simulink model "rect5angles3p"  (Simulink 7.4)
settings: Solver=ode45  StartTime=0.0  StopTime=0.08  RelTol=1e-3
undefined symbols (not defined in the file or in its folder): DiscIntNeverNeededParam, Ts
libraries: powerlib x23, powerlib_extras x1
settings Model: Creator=Safano  LastModifiedBy=ELMAY

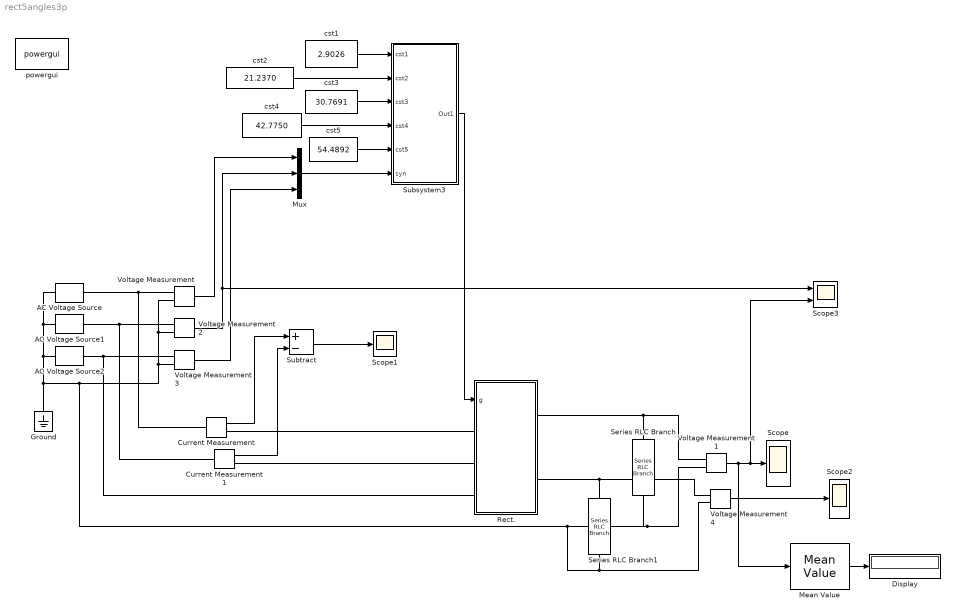
== system rect5angles3p ==
  AC Voltage Source : powerlib/Electrical Sources/AC Voltage Source  DialogController=POWERSYS.PowerSysDialog  SystemSampleTime=-1  Amplitude=220  Phase=0  Frequency=50  SampleTime=0  Measurements=None
  AC Voltage Source1 : powerlib/Electrical Sources/AC Voltage Source  DialogController=POWERSYS.PowerSysDialog  SystemSampleTime=-1  Amplitude=220  Phase=-120  Frequency=50  SampleTime=0  Measurements=None
  AC Voltage Source2 : powerlib/Electrical Sources/AC Voltage Source  DialogController=POWERSYS.PowerSysDialog  SystemSampleTime=-1  Amplitude=220  Phase=+120  Frequency=50  SampleTime=0  Measurements=None
  Current Measurement : powerlib/Measurements/Current Measurement  DialogController=POWERSYS.PowerSysDialog  SystemSampleTime=-1  PhasorSimulation=off  OutputType=Complex  PSBequivalent=0
  Current Measurement1 : powerlib/Measurements/Current Measurement  DialogController=POWERSYS.PowerSysDialog  SystemSampleTime=-1  PhasorSimulation=off  OutputType=Complex  PSBequivalent=0
  Display : Display
  Ground : powerlib/Elements/Ground  DialogController=POWERSYS.PowerSysDialog  PhysicalDomain=powersysdomain  SubClassName=unknown  LeftPortType=p1  RightPortType=p1  LConnTagsString=a
  Mean Value : powerlib_extras/Measurements/Mean Value  DialogController=POWERSYS.PowerSysDialog  SystemSampleTime=-1  Period=1/50
  Mux : Mux  Inputs=3
  Rect. : Subsystem
  Scope : Scope
      settings: SaveName=outrect
  Scope1 : Scope
  Scope2 : Scope
      settings: SaveName=outneg
  Scope3 : Scope  NumInputPorts=2
      settings: YMin=-5~-5  YMax=5~5  SaveName=crt1
  Series RLC Branch : powerlib/Elements/Series RLC Branch  DialogController=POWERSYS.PowerSysDialog  PhysicalDomain=powersysdomain  SubClassName=unknown  LeftPortType=p1  RightPortType=p1  LConnTagsString=__new0  RConnTagsString=__new0  BranchType=R  Resistance=0.3  Inductance=51e-3  SetiL0=off  InitialCurrent=0  Capacitance=1e-6  Setx0=off  InitialVoltage=0  Measurements=None
  Series RLC Branch1 : powerlib/Elements/Series RLC Branch  DialogController=POWERSYS.PowerSysDialog  PhysicalDomain=powersysdomain  SubClassName=unknown  LeftPortType=p1  RightPortType=p1  LConnTagsString=__new0  RConnTagsString=__new0  BranchType=R  Resistance=0.3  Inductance=15e-3  SetiL0=off  InitialCurrent=0  Capacitance=1e-6  Setx0=off  InitialVoltage=0  Measurements=None
  Subsystem3 : Subsystem
  Subtract : Sum  Inputs=+-  OutDataType=fixdt(1, 16)  OutScaling=2^-10
  Voltage Measurement{,1..4} (5 alike) : powerlib/Measurements/Voltage Measurement  DialogController=POWERSYS.PowerSysDialog  SystemSampleTime=-1  PhasorSimulation=off  OutputType=Complex  PSBequivalent=0
  cst1 : Constant  Value=2.9026  OutDataType=fixdt(1, 16)  OutScaling=2^0
  cst2 : Constant  Value=21.2370  OutDataType=fixdt(1, 16)  OutScaling=2^0
  cst3 : Constant  Value=30.7691  OutDataType=fixdt(1, 16)  OutScaling=2^0
  cst4 : Constant  Value=42.7750  OutDataType=fixdt(1, 16)  OutScaling=2^0
  cst5 : Constant  Value=54.4892  OutDataType=fixdt(1, 16)  OutScaling=2^0
  powergui : powerlib/powergui  Priority=1  SystemSampleTime=-1  SimulationMode=Discrete  SampleTime=50e-6  frequency=60  SPID=off  DisableSnubberDevices=off  DisableRonSwitches=off  DisableVfSwitches=off  SwTol=0  Interpol=off  frequencyindice=50  echomessages=off  HookPort=off  DisplayEquations=off  FunctionMessages=off  EnableUseOfTLC=off  x0status=blocks  RestoreLinks=warning  Frange=[0:2:500]  Ylog=off  Xlog=on  ShowGrid=off  save=off  variable=ZData  structure=outneg  ZoomFFT=off  StartTime=0.0  cycles=8  DisplayStyle=1  fundamental=150  FreqAxis=off  MaxFrequency=1000  frequencyindicesteady=1  RmsSteady=1  display=off  Ts=0  methode=off
  wires:
  cst1/1 -> Subsystem3/1(cst1)
  cst2/1 -> Subsystem3/2(cst2)
  cst3/1 -> Subsystem3/3(cst3)
  cst4/1 -> Subsystem3/4(cst4)
  cst5/1 -> Subsystem3/5(cst5)
  Mux/1 -> Subsystem3/6(syn)
  Voltage Measurement/1 -> Mux/1
  Voltage Measurement2/1 -> Mux/2, Scope3/1
  Voltage Measurement3/1 -> Mux/3
  Current Measurement/1 -> Subtract/1
  Current Measurement1/1 -> Subtract/2
  Subtract/1 -> Scope1/1
  Subsystem3/1(Out1) -> Rect./1(g)
  Voltage Measurement1/1 -> Scope/1, Scope3/2, Mean Value/1
  Voltage Measurement4/1 -> Scope2/1
  Mean Value/1 -> Display/1
  connections:
  Voltage Measurement/LConn1 -- AC Voltage Source/RConn1 -- Current Measurement/LConn1
  Voltage Measurement2/LConn1 -- AC Voltage Source1/RConn1 -- Current Measurement1/LConn1
  AC Voltage Source2/RConn1 -- Voltage Measurement3/LConn1 -- Rect./LConn3
  Current Measurement/RConn1 -- Rect./LConn1
  Voltage Measurement4/LConn2 -- Series RLC Branch1/RConn1 -- Voltage Measurement/LConn2 -- Voltage Measurement2/LConn2 -- Voltage Measurement3/LConn2 -- AC Voltage Source/LConn1 -- AC Voltage Source1/LConn1 -- AC Voltage Source2/LConn1 -- Ground/LConn1 -- Voltage Measurement1/LConn2 -- Series RLC Branch/RConn1
  Current Measurement1/RConn1 -- Rect./LConn2
  Rect./RConn1 -- Voltage Measurement1/LConn1 -- Series RLC Branch/LConn1
  Series RLC Branch1/LConn1 -- Rect./RConn2 -- Voltage Measurement4/LConn1

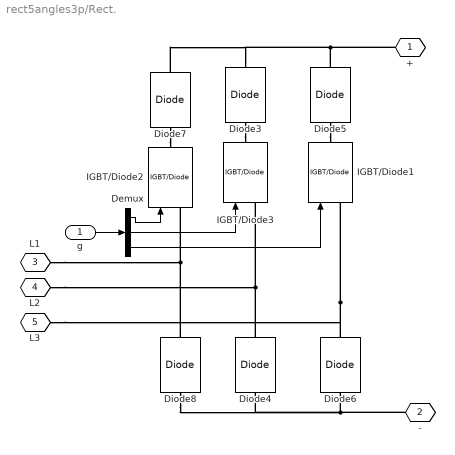
== system rect5angles3p/Rect. ==
  g : Inport  OutDataType=fixdt(1, 16)  OutScaling=2^0
  Demux : Demux  Outputs=3
  Diode{3..8} (6 alike) : powerlib/Power Electronics/Diode  DialogController=POWERSYS.PowerSysDialog  SystemSampleTime=-1  Ron=0.001  Lon=0  Vf=0.8  IC=0  UseSnubber=off  Rs=500  Cs=250e-9  Measurements=off
  IGBT/Diode1 : powerlib/Power Electronics/IGBT//Diode  DialogController=POWERSYS.PowerSysDialog  SystemSampleTime=-1  Ron=1e-3  Rs=1e5  Cs=inf  Measurements=off
  IGBT/Diode2 : powerlib/Power Electronics/IGBT//Diode  DialogController=POWERSYS.PowerSysDialog  SystemSampleTime=-1  Ron=1e-3  Rs=1e5  Cs=inf  Measurements=off
  IGBT/Diode3 : powerlib/Power Electronics/IGBT//Diode  DialogController=POWERSYS.PowerSysDialog  SystemSampleTime=-1  Ron=1e-3  Rs=1e5  Cs=inf  Measurements=off
  + : PMIOPort  Tag=PMCPort  Port=1  Side=Right
  - : PMIOPort  Tag=PMCPort  Port=2  Side=Right
  L1 : PMIOPort  Tag=PMCPort  Port=3  Side=Left
  L2 : PMIOPort  Tag=PMCPort  Port=4  Side=Left
  L3 : PMIOPort  Tag=PMCPort  Port=5  Side=Left
  wires:
  Demux/1 -> IGBT/Diode2/1
  Demux/2 -> IGBT/Diode3/1
  Demux/3 -> IGBT/Diode1/1
  g/1 -> Demux/1
  connections:
  Diode3/LConn1 -- IGBT/Diode3/RConn1
  +/RConn1 -- Diode5/RConn1 -- Diode7/RConn1 -- Diode3/RConn1
  -/RConn1 -- Diode8/LConn1 -- Diode4/LConn1 -- Diode6/LConn1
  L2/RConn1 -- Diode4/RConn1 -- IGBT/Diode3/LConn1
  Diode5/LConn1 -- IGBT/Diode1/RConn1
  L3/RConn1 -- Diode6/RConn1 -- IGBT/Diode1/LConn1
  Diode7/LConn1 -- IGBT/Diode2/RConn1
  L1/RConn1 -- Diode8/RConn1 -- IGBT/Diode2/LConn1

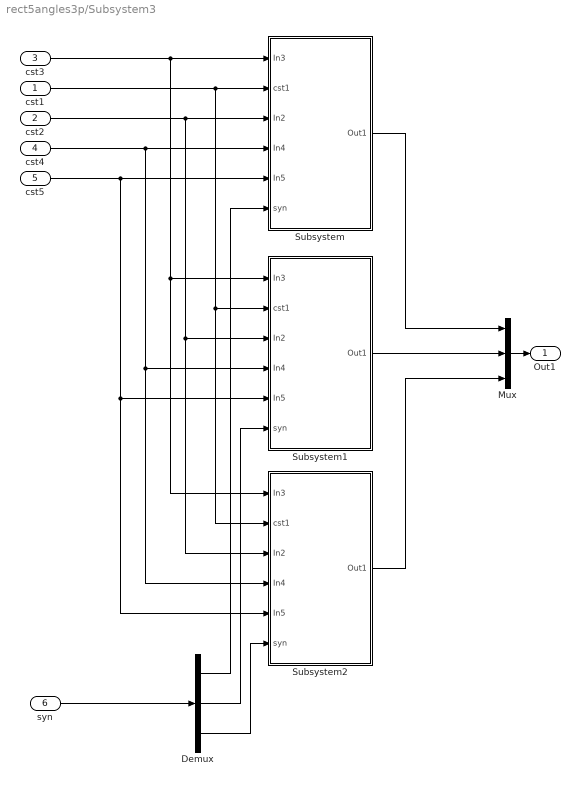
== system rect5angles3p/Subsystem3 ==
  cst1 : Inport  OutDataType=fixdt(1, 16)  OutScaling=2^0
  cst2 : Inport  Port=2  OutDataType=fixdt(1, 16)  OutScaling=2^0
  cst3 : Inport  Port=3  OutDataType=fixdt(1, 16)  OutScaling=2^0
  cst4 : Inport  Port=4  OutDataType=fixdt(1, 16)  OutScaling=2^0
  cst5 : Inport  Port=5  OutDataType=fixdt(1, 16)  OutScaling=2^0
  syn : Inport  Port=6  OutDataType=fixdt(1, 16)  OutScaling=2^0
  Demux : Demux  Outputs=3
  Mux : Mux  Inputs=3
  Subsystem : Subsystem
  Subsystem1 : Subsystem
  Subsystem2 : Subsystem
  Out1 : Outport  OutDataType=fixdt(1, 16)  OutScaling=2^0
  wires:
  Subsystem1/1(Out1) -> Mux/2
  Subsystem/1(Out1) -> Mux/1
  Subsystem2/1(Out1) -> Mux/3
  Demux/3 -> Subsystem2/6(syn)
  Demux/2 -> Subsystem1/6(syn)
  Demux/1 -> Subsystem/6(syn)
  cst1/1 -> Subsystem/2(cst1), Subsystem1/2(cst1), Subsystem2/2(cst1)
  cst2/1 -> Subsystem/3(In2), Subsystem1/3(In2), Subsystem2/3(In2)
  cst3/1 -> Subsystem/1(In3), Subsystem1/1(In3), Subsystem2/1(In3)
  cst4/1 -> Subsystem/4(In4), Subsystem1/4(In4), Subsystem2/4(In4)
  cst5/1 -> Subsystem/5(In5), Subsystem2/5(In5), Subsystem1/5(In5)
  syn/1 -> Demux/1
  Mux/1 -> Out1/1

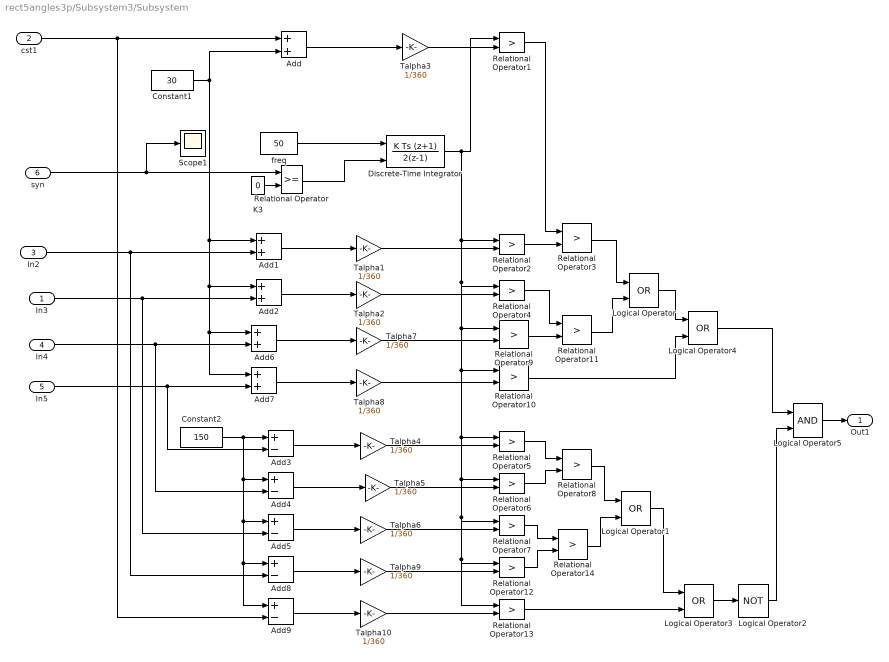
== system rect5angles3p/Subsystem3/Subsystem ==
  In3 : Inport  OutDataType=fixdt(1, 16)  OutScaling=2^0
  cst1 : Inport  Port=2  OutDataType=fixdt(1, 16)  OutScaling=2^0
  In2 : Inport  Port=3  OutDataType=fixdt(1, 16)  OutScaling=2^0
  In4 : Inport  Port=4  OutDataType=fixdt(1, 16)  OutScaling=2^0
  In5 : Inport  Port=5  OutDataType=fixdt(1, 16)  OutScaling=2^0
  syn : Inport  Port=6  OutDataType=fixdt(1, 16)  OutScaling=2^0
  Add{,1..2,6..7} (5 alike) : Sum  OutDataType=fixdt(1, 16)  OutScaling=2^-10
  Add{3..5,8..9} (5 alike) : Sum  Inputs=+-  OutDataType=fixdt(1, 16)  OutScaling=2^-10
  Constant1 : Constant  Value=30  OutDataType=fixdt(1, 16)  OutScaling=2^0
  Constant2 : Constant  Value=150  OutDataType=fixdt(1, 16)  OutScaling=2^0
  Discrete-Time Integrator : DiscreteIntegrator  IntegratorMethod=Integration: Trapezoidal  ExternalReset=rising  InitialConditionMode=State only (most efficient)  SampleTime=Ts  OutDataType=sfix(16)  OutScaling=2^0  ICPrevOutput=DiscIntNeverNeededParam  ICPrevScaledInput=DiscIntNeverNeededParam
  K3 : Constant  Value=0  OutDataType=sfix(16)  OutScaling=2^0
  Logical Operator{,1,3..4} (4 alike) : Logic  Operator=OR  AllPortsSameDT=off  OutDataTypeMode=boolean  LogicDataType=fixdt(0, 8)  OutDataTypeStr=boolean
  Logical Operator2 : Logic  Operator=NOT  AllPortsSameDT=off  OutDataTypeMode=boolean  LogicDataType=fixdt(0, 8)  OutDataTypeStr=boolean
  Logical Operator5 : Logic  AllPortsSameDT=off  OutDataTypeMode=boolean  LogicDataType=fixdt(0, 8)  OutDataTypeStr=boolean
  Relational Operator : RelationalOperator  InputSameDT=on
  Relational Operator{1..14} (14 alike) : RelationalOperator  Operator=>  InputSameDT=on
  Scope1 : Scope
      settings: SaveName=ScopeData2
  Talpha{1..10} (10 alike) : Gain  Gain=1/360  ParameterDataType=sfix(16)  ParameterScaling=2^0  OutDataType=sfix(16)  OutScaling=2^0  SaturateOnIntegerOverflow=on  OutDataTypeStr=Inherit: Same as input  ParamDataTypeStr=Inherit: Same as input
  freq : Constant  Value=50  OutDataType=sfix(16)  OutScaling=2^0
  Out1 : Outport  OutDataType=fixdt(1, 16)  OutScaling=2^0
  wires:
  Relational Operator1/1 -> Relational Operator3/1
  Discrete-Time Integrator/1 -> Relational Operator2/1, Relational Operator4/1, Relational Operator9/1, Relational Operator5/1, Relational Operator6/1, Relational Operator7/1, Relational Operator12/1, Relational Operator13/1, Relational Operator10/1, Relational Operator1/1
  Talpha3/1 -> Relational Operator1/2
  freq/1 -> Discrete-Time Integrator/1
  Talpha1/1 -> Relational Operator2/2
  K3/1 -> Relational Operator/2
  Relational Operator/1 -> Discrete-Time Integrator/2
  syn/1 -> Relational Operator/1, Scope1/1
  Talpha2/1 -> Relational Operator4/2
  Add2/1 -> Talpha2/1
  Relational Operator4/1 -> Relational Operator11/1
  Logical Operator/1 -> Logical Operator4/1
  Relational Operator3/1 -> Logical Operator/1
  Relational Operator2/1 -> Relational Operator3/2
  Talpha4/1 -> Relational Operator5/2
  Add3/1 -> Talpha4/1
  Talpha5/1 -> Relational Operator6/2
  Talpha6/1 -> Relational Operator7/2
  Relational Operator5/1 -> Relational Operator8/1
  Relational Operator6/1 -> Relational Operator8/2
  Relational Operator8/1 -> Logical Operator1/1
  Add/1 -> Talpha3/1
  cst1/1 -> Add/1, Add9/2
  Constant1/1 -> Add/2, Add1/1, Add2/1, Add6/1, Add7/1
  Add1/1 -> Talpha1/1
  In2/1 -> Add1/2, Add8/2
  In3/1 -> Add2/2, Add5/2
  Add5/1 -> Talpha6/1
  Add4/1 -> Talpha5/1
  Constant2/1 -> Add3/1, Add4/1, Add5/1, Add8/1, Add9/1
  In4/1 -> Add6/2, Add4/2
  In5/1 -> Add7/2, Add3/2
  Add6/1 -> Talpha7/1
  Add7/1 -> Talpha8/1
  Talpha7/1 -> Relational Operator9/2
  Talpha8/1 -> Relational Operator10/2
  Relational Operator9/1 -> Relational Operator11/2
  Relational Operator11/1 -> Logical Operator/2
  Relational Operator10/1 -> Logical Operator4/2
  Add8/1 -> Talpha9/1
  Add9/1 -> Talpha10/1
  Talpha9/1 -> Relational Operator12/2
  Talpha10/1 -> Relational Operator13/2
  Relational Operator12/1 -> Relational Operator14/2
  Relational Operator7/1 -> Relational Operator14/1
  Relational Operator14/1 -> Logical Operator1/2
  Relational Operator13/1 -> Logical Operator3/2
  Logical Operator1/1 -> Logical Operator3/1
  Logical Operator3/1 -> Logical Operator2/1
  Logical Operator4/1 -> Logical Operator5/1
  Logical Operator2/1 -> Logical Operator5/2
  Logical Operator5/1 -> Out1/1

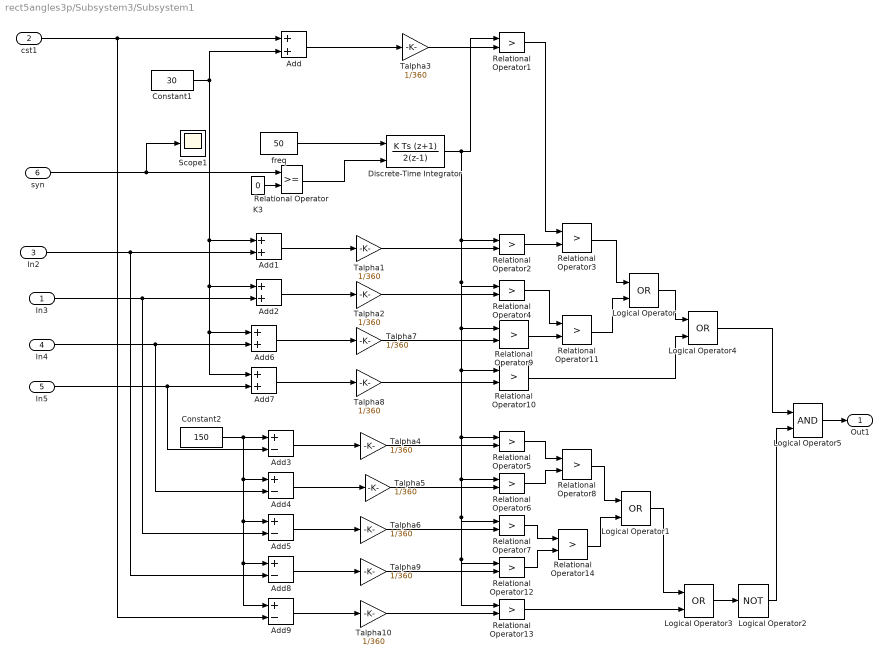
== system rect5angles3p/Subsystem3/Subsystem1 ==
  In3 : Inport  OutDataType=fixdt(1, 16)  OutScaling=2^0
  cst1 : Inport  Port=2  OutDataType=fixdt(1, 16)  OutScaling=2^0
  In2 : Inport  Port=3  OutDataType=fixdt(1, 16)  OutScaling=2^0
  In4 : Inport  Port=4  OutDataType=fixdt(1, 16)  OutScaling=2^0
  In5 : Inport  Port=5  OutDataType=fixdt(1, 16)  OutScaling=2^0
  syn : Inport  Port=6  OutDataType=fixdt(1, 16)  OutScaling=2^0
  Add{,1..2,6..7} (5 alike) : Sum  OutDataType=fixdt(1, 16)  OutScaling=2^-10
  Add{3..5,8..9} (5 alike) : Sum  Inputs=+-  OutDataType=fixdt(1, 16)  OutScaling=2^-10
  Constant1 : Constant  Value=30  OutDataType=fixdt(1, 16)  OutScaling=2^0
  Constant2 : Constant  Value=150  OutDataType=fixdt(1, 16)  OutScaling=2^0
  Discrete-Time Integrator : DiscreteIntegrator  IntegratorMethod=Integration: Trapezoidal  ExternalReset=rising  InitialConditionMode=State only (most efficient)  SampleTime=Ts  OutDataType=sfix(16)  OutScaling=2^0  ICPrevOutput=DiscIntNeverNeededParam  ICPrevScaledInput=DiscIntNeverNeededParam
  K3 : Constant  Value=0  OutDataType=sfix(16)  OutScaling=2^0
  Logical Operator{,1,3..4} (4 alike) : Logic  Operator=OR  AllPortsSameDT=off  OutDataTypeMode=boolean  LogicDataType=fixdt(0, 8)  OutDataTypeStr=boolean
  Logical Operator2 : Logic  Operator=NOT  AllPortsSameDT=off  OutDataTypeMode=boolean  LogicDataType=fixdt(0, 8)  OutDataTypeStr=boolean
  Logical Operator5 : Logic  AllPortsSameDT=off  OutDataTypeMode=boolean  LogicDataType=fixdt(0, 8)  OutDataTypeStr=boolean
  Relational Operator : RelationalOperator  InputSameDT=on
  Relational Operator{1..14} (14 alike) : RelationalOperator  Operator=>  InputSameDT=on
  Scope1 : Scope
      settings: SaveName=ScopeData2
  Talpha{1..10} (10 alike) : Gain  Gain=1/360  ParameterDataType=sfix(16)  ParameterScaling=2^0  OutDataType=sfix(16)  OutScaling=2^0  SaturateOnIntegerOverflow=on  OutDataTypeStr=Inherit: Same as input  ParamDataTypeStr=Inherit: Same as input
  freq : Constant  Value=50  OutDataType=sfix(16)  OutScaling=2^0
  Out1 : Outport  OutDataType=fixdt(1, 16)  OutScaling=2^0
  wires:
  Logical Operator5/1 -> Out1/1
  Logical Operator2/1 -> Logical Operator5/2
  Logical Operator4/1 -> Logical Operator5/1
  Logical Operator3/1 -> Logical Operator2/1
  Logical Operator1/1 -> Logical Operator3/1
  Relational Operator13/1 -> Logical Operator3/2
  Relational Operator14/1 -> Logical Operator1/2
  Relational Operator7/1 -> Relational Operator14/1
  Relational Operator12/1 -> Relational Operator14/2
  Talpha10/1 -> Relational Operator13/2
  Talpha9/1 -> Relational Operator12/2
  Add9/1 -> Talpha10/1
  Add8/1 -> Talpha9/1
  Relational Operator10/1 -> Logical Operator4/2
  Relational Operator11/1 -> Logical Operator/2
  Relational Operator9/1 -> Relational Operator11/2
  Talpha8/1 -> Relational Operator10/2
  Talpha7/1 -> Relational Operator9/2
  Add7/1 -> Talpha8/1
  Add6/1 -> Talpha7/1
  In5/1 -> Add3/2, Add7/2
  In4/1 -> Add4/2, Add6/2
  Constant2/1 -> Add9/1, Add8/1, Add5/1, Add4/1, Add3/1
  Add4/1 -> Talpha5/1
  Add5/1 -> Talpha6/1
  In3/1 -> Add5/2, Add2/2
  In2/1 -> Add8/2, Add1/2
  Add1/1 -> Talpha1/1
  Constant1/1 -> Add7/1, Add6/1, Add2/1, Add1/1, Add/2
  cst1/1 -> Add9/2, Add/1
  Add/1 -> Talpha3/1
  Relational Operator8/1 -> Logical Operator1/1
  Relational Operator6/1 -> Relational Operator8/2
  Relational Operator5/1 -> Relational Operator8/1
  Talpha6/1 -> Relational Operator7/2
  Talpha5/1 -> Relational Operator6/2
  Add3/1 -> Talpha4/1
  Talpha4/1 -> Relational Operator5/2
  Relational Operator2/1 -> Relational Operator3/2
  Relational Operator3/1 -> Logical Operator/1
  Logical Operator/1 -> Logical Operator4/1
  Relational Operator4/1 -> Relational Operator11/1
  Add2/1 -> Talpha2/1
  Talpha2/1 -> Relational Operator4/2
  syn/1 -> Scope1/1, Relational Operator/1
  Relational Operator/1 -> Discrete-Time Integrator/2
  K3/1 -> Relational Operator/2
  Talpha1/1 -> Relational Operator2/2
  freq/1 -> Discrete-Time Integrator/1
  Talpha3/1 -> Relational Operator1/2
  Discrete-Time Integrator/1 -> Relational Operator1/1, Relational Operator10/1, Relational Operator13/1, Relational Operator12/1, Relational Operator7/1, Relational Operator6/1, Relational Operator5/1, Relational Operator9/1, Relational Operator4/1, Relational Operator2/1
  Relational Operator1/1 -> Relational Operator3/1

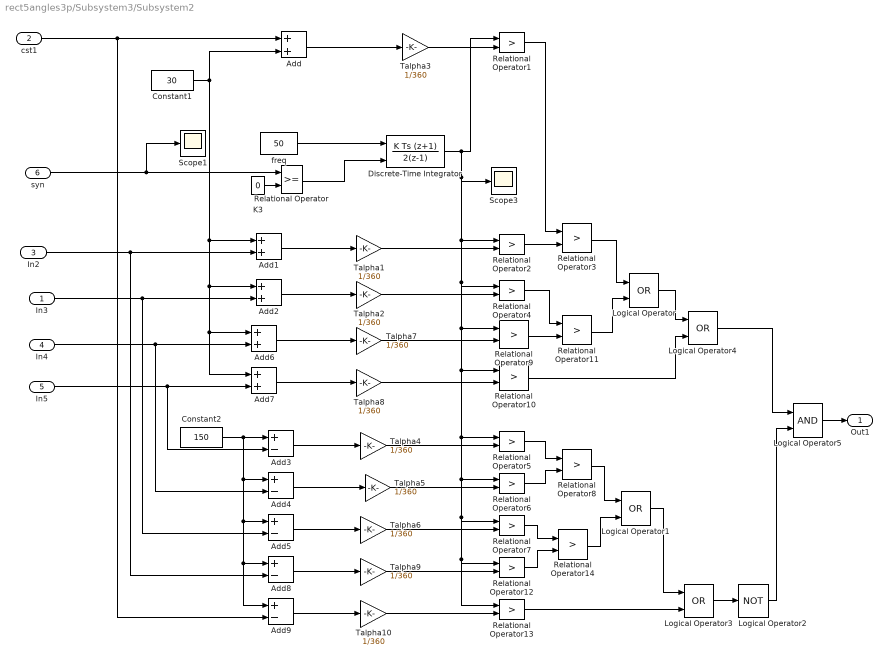
== system rect5angles3p/Subsystem3/Subsystem2 ==
  In3 : Inport  OutDataType=fixdt(1, 16)  OutScaling=2^0
  cst1 : Inport  Port=2  OutDataType=fixdt(1, 16)  OutScaling=2^0
  In2 : Inport  Port=3  OutDataType=fixdt(1, 16)  OutScaling=2^0
  In4 : Inport  Port=4  OutDataType=fixdt(1, 16)  OutScaling=2^0
  In5 : Inport  Port=5  OutDataType=fixdt(1, 16)  OutScaling=2^0
  syn : Inport  Port=6  OutDataType=fixdt(1, 16)  OutScaling=2^0
  Add{,1..2,6..7} (5 alike) : Sum  OutDataType=fixdt(1, 16)  OutScaling=2^-10
  Add{3..5,8..9} (5 alike) : Sum  Inputs=+-  OutDataType=fixdt(1, 16)  OutScaling=2^-10
  Constant1 : Constant  Value=30  OutDataType=fixdt(1, 16)  OutScaling=2^0
  Constant2 : Constant  Value=150  OutDataType=fixdt(1, 16)  OutScaling=2^0
  Discrete-Time Integrator : DiscreteIntegrator  IntegratorMethod=Integration: Trapezoidal  ExternalReset=rising  InitialConditionMode=State only (most efficient)  SampleTime=Ts  OutDataType=sfix(16)  OutScaling=2^0  ICPrevOutput=DiscIntNeverNeededParam  ICPrevScaledInput=DiscIntNeverNeededParam
  K3 : Constant  Value=0  OutDataType=sfix(16)  OutScaling=2^0
  Logical Operator{,1,3..4} (4 alike) : Logic  Operator=OR  AllPortsSameDT=off  OutDataTypeMode=boolean  LogicDataType=fixdt(0, 8)  OutDataTypeStr=boolean
  Logical Operator2 : Logic  Operator=NOT  AllPortsSameDT=off  OutDataTypeMode=boolean  LogicDataType=fixdt(0, 8)  OutDataTypeStr=boolean
  Logical Operator5 : Logic  AllPortsSameDT=off  OutDataTypeMode=boolean  LogicDataType=fixdt(0, 8)  OutDataTypeStr=boolean
  Relational Operator : RelationalOperator  InputSameDT=on
  Relational Operator{1..14} (14 alike) : RelationalOperator  Operator=>  InputSameDT=on
  Scope1 : Scope
      settings: SaveName=ScopeData2
  Scope3 : Scope
      settings: SaveName=ScopeData7
  Talpha{1..10} (10 alike) : Gain  Gain=1/360  ParameterDataType=sfix(16)  ParameterScaling=2^0  OutDataType=sfix(16)  OutScaling=2^0  SaturateOnIntegerOverflow=on  OutDataTypeStr=Inherit: Same as input  ParamDataTypeStr=Inherit: Same as input
  freq : Constant  Value=50  OutDataType=sfix(16)  OutScaling=2^0
  Out1 : Outport  OutDataType=fixdt(1, 16)  OutScaling=2^0
  wires:
  Logical Operator5/1 -> Out1/1
  Logical Operator2/1 -> Logical Operator5/2
  Logical Operator4/1 -> Logical Operator5/1
  Logical Operator3/1 -> Logical Operator2/1
  Logical Operator1/1 -> Logical Operator3/1
  Relational Operator13/1 -> Logical Operator3/2
  Relational Operator14/1 -> Logical Operator1/2
  Relational Operator7/1 -> Relational Operator14/1
  Relational Operator12/1 -> Relational Operator14/2
  Talpha10/1 -> Relational Operator13/2
  Talpha9/1 -> Relational Operator12/2
  Add9/1 -> Talpha10/1
  Add8/1 -> Talpha9/1
  Relational Operator10/1 -> Logical Operator4/2
  Relational Operator11/1 -> Logical Operator/2
  Relational Operator9/1 -> Relational Operator11/2
  Talpha8/1 -> Relational Operator10/2
  Talpha7/1 -> Relational Operator9/2
  Add7/1 -> Talpha8/1
  Add6/1 -> Talpha7/1
  In5/1 -> Add3/2, Add7/2
  In4/1 -> Add4/2, Add6/2
  Constant2/1 -> Add9/1, Add8/1, Add5/1, Add4/1, Add3/1
  Add4/1 -> Talpha5/1
  Add5/1 -> Talpha6/1
  In3/1 -> Add5/2, Add2/2
  In2/1 -> Add8/2, Add1/2
  Add1/1 -> Talpha1/1
  Constant1/1 -> Add7/1, Add6/1, Add2/1, Add1/1, Add/2
  cst1/1 -> Add9/2, Add/1
  Add/1 -> Talpha3/1
  Relational Operator8/1 -> Logical Operator1/1
  Relational Operator6/1 -> Relational Operator8/2
  Relational Operator5/1 -> Relational Operator8/1
  Talpha6/1 -> Relational Operator7/2
  Talpha5/1 -> Relational Operator6/2
  Add3/1 -> Talpha4/1
  Talpha4/1 -> Relational Operator5/2
  Relational Operator2/1 -> Relational Operator3/2
  Relational Operator3/1 -> Logical Operator/1
  Logical Operator/1 -> Logical Operator4/1
  Relational Operator4/1 -> Relational Operator11/1
  Add2/1 -> Talpha2/1
  Talpha2/1 -> Relational Operator4/2
  syn/1 -> Scope1/1, Relational Operator/1
  Relational Operator/1 -> Discrete-Time Integrator/2
  K3/1 -> Relational Operator/2
  Talpha1/1 -> Relational Operator2/2
  freq/1 -> Discrete-Time Integrator/1
  Talpha3/1 -> Relational Operator1/2
  Discrete-Time Integrator/1 -> Relational Operator1/1, Relational Operator10/1, Relational Operator13/1, Relational Operator12/1, Relational Operator7/1, Relational Operator6/1, Relational Operator5/1, Relational Operator9/1, Relational Operator4/1, Relational Operator2/1, Scope3/1
  Relational Operator1/1 -> Relational Operator3/1
